simulink model "My_gfm_datacenter_BESS"  (R2018b)
settings: Solver=ode45  StartTime=0.0  StopTime=100  MaxStep=1e-4  RelTol=1e-3
PreLoadFcn:
  | modelDir = fileparts(get_param(bdroot,'FileName'));
  | 
  | load_system(fullfile(modelDir,'controls_element_lib.slx'));
  | load_system(fullfile(modelDir,'test_sequence_lib.slx'));
InitFcn:
  | close all;
  | clear all;
  | clc;
  | 
  | close all;
  | clear all;
  | clc;
  | 
  | % frequency nominals
  | F_NOM = 60;
  | W_NOM = 2 * pi * F_NOM;
  | 
  | % base values relative to inverter
  | % --------------------------------
  | VLL_INV_NOM = 34.5e3;
  | P_INV_NOM = 5e6;
  | Q_INV_NOM = 2.5e6;
  | S_INV_NOM = sqrt(P_INV_NOM^2 + Q_INV_NOM^2);
  | 
  | I_INV_BASE = S_INV_NOM/(sqrt(3)*VLL_INV_NOM);
  | Z_INV_BASE = VLL_INV_NOM^2/S_INV_NOM;
  | L_INV_BASE = Z_INV_BASE / W_NOM;
  | C_INV_BASE = 1 / (Z_INV_BASE * W_NOM);
  | 
  | % SST Parameters
  | N_DCDC_XFMR = 3;
  | N_CELLS_PER_STRING = 10;
  | C_MV_CELL = 400e-6;
  | C_LV_SST = 5e-3;
  | C_BBU = 1500; % 60 sec * 5MW
  | r_BBU = 5e-3;
  | ILV_MAX = 300;
  | ILV_MIN = -300;
  | IMV_MAX = 100;
  | IMV_MIN = -100;
  | V_LVDC_NOM = 800;
  | IDC_NOM = P_INV_NOM / V_LVDC_NOM;
  | 
  | % nominal ratings for power system model
  | % --------------------------------------
  | INVERTER_COUNT = 20;
  | 
  | VMV_NOM = VLL_INV_NOM;
  | VHV_NOM = 230e3;
  | S_PLANT = INVERTER_COUNT * S_INV_NOM;
  | 
  | N_GSU = VHV_NOM/VMV_NOM;
  | 
  | I_MV_BASE = S_PLANT/(sqrt(3)*VMV_NOM);
  | I_HV_BASE = S_PLANT/(sqrt(3)*VHV_NOM);
  | 
  | Z_MV_BASE = VMV_NOM^2/S_PLANT;
  | Z_HV_BASE = VHV_NOM^2/S_PLANT;
  | 
  | L_MV_BASE = Z_MV_BASE / W_NOM;
  | L_HV_BASE = Z_HV_BASE / W_NOM;
  | C_MV_BASE = 1 / (Z_MV_BASE * W_NOM);
  | C_HV_BASE = 1 / (Z_HV_BASE * W_NOM);
libraries: controls_element_lib x20, test_sequence_lib x13, simulink x3
settings Model: SimulationMode=accelerator  Creator=HussamAlatrash  LastModifiedBy=ahhei
settings DataIOCC: SaveOutput=off  SignalLogging=off  DSMLogging=off  SaveTime=off
settings OptimizationCC: EfficientMapNaN2IntZero=off
settings DebuggingCC: UnconnectedInputMsg=none  UnconnectedOutputMsg=none  UnconnectedLineMsg=none
settings HardwareCC: TargetBitPerPointer=64  TargetBitPerSizeT=64  TargetBitPerPtrDiffT=64  TargetLongLongMode=on  TargetIntDivRoundTo=Zero  TargetEndianess=LittleEndian  TargetWordSize=64  TargetHWDeviceType=MATLAB Host  ProdEqTarget=off
settings ModelReferenceCC: EnableRefExpFcnMdlSchedulingChecks=off
settings CodeAppCC: MaxIdLength=128
settings GRTTargetCC: TargetLangStandard=C89/C90 (ANSI)  CombineOutputUpdateFcns=off  GRTInterface=on

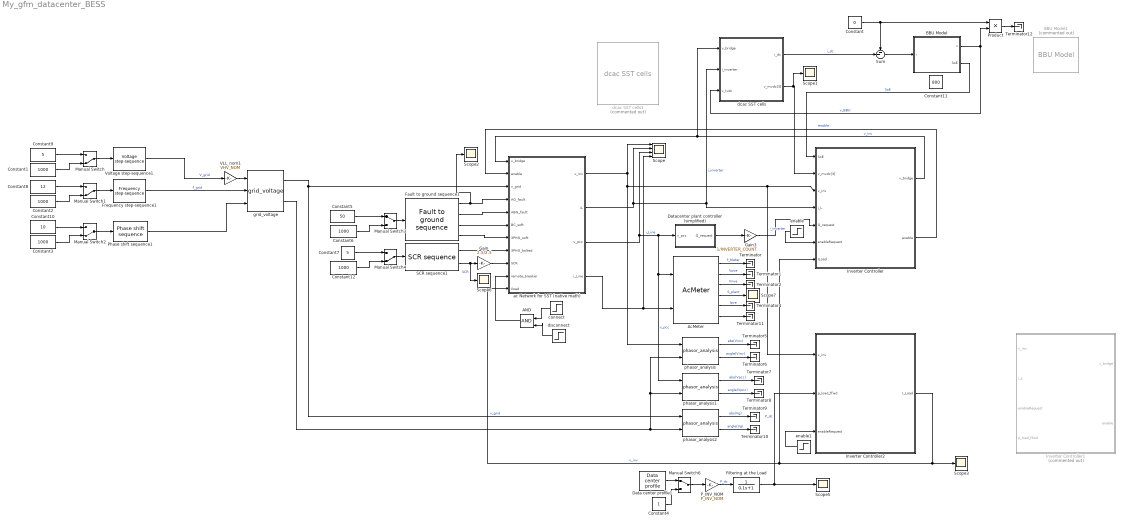
== system My_gfm_datacenter_BESS ==
  AND : Logic  IconShape=distinctive  AllPortsSameDT=off  OutDataTypeStr=boolean
  AcMeter : test_sequence_lib/AcMeter  VllRated=VHV_NOM
  BBU Model : Subsystem  AncestorBlock=test_sequence_lib/BBU Model
  BBU Model1 : test_sequence_lib/BBU Model  Commented=on  SystemSampleTime=-1
  Constant : Constant  Value=0
  Constant{1..3,6,12} (5 alike) : Constant  Value=1000
  Constant10 : Constant  Value=10
  Constant11 : Constant  Value=800
  Constant4 : Constant
  Constant5 : Constant  Value=50
  Constant7 : Constant  Value=5
  Constant8 : Constant  Value=12
  Constant9 : Constant  Value=5
  Data center profile1 : test_sequence_lib/Data center profile  SystemSampleTime=-1
  Datacenter plant controller (simplified) : Subsystem  AncestorBlock=controls_element_lib/Datacenter plant controller
  Fault to ground sequence1 : test_sequence_lib/Fault to ground sequence  SystemSampleTime=-1
  Filtering at the Load : TransferFcn  Denominator=[0.1 1]
  Frequency step-sequence1 : test_sequence_lib/Frequency step-sequence  SystemSampleTime=-1
  Gain : Gain  Gain=2.5/2.5
  Gain3 : Gain  Gain=1/INVERTER_COUNT
  Inverter Controller : Subsystem
  Inverter Controller1 : Subsystem  Commented=on
  Inverter Controller2 : Subsystem
  Manual Switch{,1..2,4} (4 alike) : ManualSwitch  CurrentSetting=0
  Manual Switch3 : ManualSwitch
  Manual Switch6 : ManualSwitch
  P_INV_NOM : Gain  Gain=P_INV_NOM
  Phase shift sequence1 : test_sequence_lib/Phase shift sequence  SystemSampleTime=-1
  Product : Product
  SCR sequence1 : test_sequence_lib/SCR sequence  SystemSampleTime=-1
  Scope : Scope  NumInputPorts=4
  Scope{1..3,5..7} (6 alike) : Scope
  Sum : Sum  Inputs=--|
  Terminator{,1..2,4..12} (12 alike) : Terminator
  VLL_nom1 : Gain  Gain=VHV_NOM
  Voltage step-sequence1 : test_sequence_lib/Voltage step-sequence  SystemSampleTime=-1
  ac Network for SST (native math) : Subsystem  AncestorBlock=test_sequence_lib/ac Network for SST (native math)
  connect : Step  Time=0  SampleTime=0
  dcac SST cells : Subsystem  AncestorBlock=test_sequence_lib/dcac SST cells
  dcac SST cells1 : test_sequence_lib/dcac SST cells  Commented=on  SystemSampleTime=-1
  disconnect : Step  Time=97  Before=1  SampleTime=0
  enable : Step  Time=2  SampleTime=0
  enable1 : Step  Time=4  SampleTime=0
  grid_voltage : test_sequence_lib/grid_voltage  SystemSampleTime=-1
  phasor_analysis : test_sequence_lib/phasor_analysis  SystemSampleTime=-1
  phasor_analysis1 : test_sequence_lib/phasor_analysis  SystemSampleTime=-1
  phasor_analysis2 : test_sequence_lib/phasor_analysis  SystemSampleTime=-1
  wires:
  Inverter Controller/2(enable) -> ac Network for SST (native math)/2(enable)  "enable"
  Constant9/1 -> Manual Switch/1
  Constant3/1 -> Manual Switch2/2
  VLL_nom1/1 -> grid_voltage/1
  Manual Switch3/1 -> Fault to ground sequence1/1
  Voltage step-sequence1/1 -> VLL_nom1/1  "V_grid"
  Constant6/1 -> Manual Switch3/2
  Fault to ground sequence1/2 -> ac Network for SST (native math)/5(ABG_fault)
  ac Network for SST (native math)/4(i_Line) -> Scope/4, AcMeter/2  "i_Line"
  ac Network for SST (native math)/1(v_inv) -> Scope/1, Inverter Controller2/1(v_inv), Inverter Controller/3(v_inv), phasor_analysis/1  "i_inverter"
  Constant8/1 -> Manual Switch1/1
  Gain/1 -> ac Network for SST (native math)/9(SCR)
  Inverter Controller/1(v_bridge) -> dcac SST cells/1(v_bridge), ac Network for SST (native math)/1(v_bridge)  "v_inv"
  SCR sequence1/2 -> Scope6/1, Gain/1  "SCR"
  phasor_analysis1/2 -> Terminator8/1  "angle(Vpcc)"
  Constant1/1 -> Manual Switch/2
  Fault to ground sequence1/1 -> Scope2/1, ac Network for SST (native math)/4(AG_fault)
  Frequency step-sequence1/1 -> grid_voltage/2  "f_grid"
  Constant5/1 -> Manual Switch3/1
  Fault to ground sequence1/4 -> ac Network for SST (native math)/7(3PHG_soft)
  Fault to ground sequence1/3 -> ac Network for SST (native math)/6(BC_soft)
  AcMeter/2 -> Terminator1/1  "Vpve"
  dcac SST cells/1(i_dc) -> Sum/2  "i_dc"
  phasor_analysis/1 -> Terminator5/1  "abs(Vinv)"
  AcMeter/4 -> Scope7/1  "S_plant"
  Manual Switch/1 -> Voltage step-sequence1/1
  Manual Switch1/1 -> Frequency step-sequence1/1
  Datacenter plant controller (simplified)/1(Q_request) -> Gain3/1
  connect/1 -> AND/1
  Phase shift sequence1/1 -> grid_voltage/3
  Constant10/1 -> Manual Switch2/1
  disconnect/1 -> AND/2
  ac Network for SST (native math)/2(iL) -> Scope/2, Inverter Controller/4(i_L), dcac SST cells/2(i_inverter)  "i_inverter"
  dcac SST cells/2(v_mvdc[3]) -> Scope1/1, Inverter Controller/2(v_mvdc[3])
  AND/1 -> ac Network for SST (native math)/10(remote_breaker)
  enable/1 -> Inverter Controller/6(enableRequest)
  Constant7/1 -> Manual Switch4/1
  grid_voltage/2 -> phasor_analysis1/2, phasor_analysis/2, phasor_analysis2/2
  grid_voltage/1 -> phasor_analysis2/1, ac Network for SST (native math)/3(v_grid)  "v_grid"
  SCR sequence1/1 -> ac Network for SST (native math)/8(3PHG_bolted)
  phasor_analysis1/1 -> Terminator7/1  "abs(Vpcc)"
  ac Network for SST (native math)/3(v_pcc) -> Scope/3, Datacenter plant controller (simplified)/1(v_pcc), phasor_analysis1/1, AcMeter/1  "v_pcc"
  Constant12/1 -> Manual Switch4/2
  BBU Model/1(v) -> dcac SST cells/3(v_lvdc), Product/2  "v_BBU"
  Constant/1 -> Sum/1, Product/1
  phasor_analysis2/2 -> Terminator10/1  "angle(Vg)"
  BBU Model/2(SoE) -> Inverter Controller/1(SoE)  "SoE"
  Gain3/1 -> Inverter Controller/5(Q_request)
  phasor_analysis/2 -> Terminator6/1  "angle(Vinv)"
  AcMeter/3 -> Terminator2/1  "Vnve"
  AcMeter/5 -> Terminator4/1  "Ipve"
  Constant2/1 -> Manual Switch1/2
  phasor_analysis2/1 -> Terminator9/1  "abs(Vg)"
  Manual Switch4/1 -> SCR sequence1/1
  Sum/1 -> BBU Model/1(i)
  AcMeter/6 -> Terminator11/1
  AcMeter/1 -> Terminator/1  "f_Meter"
  Manual Switch2/1 -> Phase shift sequence1/1
  enable1/1 -> Inverter Controller2/3(enableRequest)
  Inverter Controller2/1(I_Load) -> Inverter Controller/7(ILoad), ac Network for SST (native math)/11(Iload), Scope3/1  "v_inv"
  Manual Switch6/1 -> P_INV_NOM/1
  Data center profile1/1 -> Manual Switch6/1
  Constant4/1 -> Manual Switch6/2
  P_INV_NOM/1 -> Filtering at the Load/1  "P_dc"
  Product/1 -> Terminator12/1
  Filtering at the Load/1 -> Inverter Controller2/2(p_load_ffwd), Scope5/1  "P_dc"

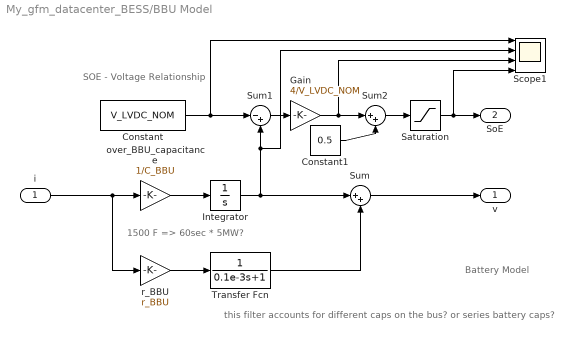
== system My_gfm_datacenter_BESS/BBU Model ==
  note: Battery Model
  note: this filter accounts for different caps on the bus? or series battery caps?
  note: 1500 F => 60sec * 5MW?
  note: SOE - Voltage Relationship
  i : Inport
  Constant : Constant  Value=V_LVDC_NOM
  Constant1 : Constant  Value=0.5
  Gain : Gain  Gain=4/V_LVDC_NOM
  Integrator : Integrator  InitialCondition=V_LVDC_NOM
  Saturation : Saturate  UpperLimit=1.1  LowerLimit=-0.1
  Scope1 : Scope  NumInputPorts=4
  Sum : Sum  Inputs=|++
  Sum1 : Sum  Inputs=|-+
  Sum2 : Sum  Inputs=|++
  Transfer Fcn : TransferFcn  Denominator=[0.1e-3 1]
  over_BBU_capacitance : Gain  Gain=1/C_BBU
  r_BBU : Gain  Gain=r_BBU
  v : Outport  VectorParamsAs1DForOutWhenUnconnected=on
  SoE : Outport  Port=2  VectorParamsAs1DForOutWhenUnconnected=on
  wires:
  Saturation/1 -> Scope1/4, SoE/1
  Constant1/1 -> Sum2/2
  Sum2/1 -> Saturation/1
  Constant/1 -> Scope1/1, Sum1/1
  Sum1/1 -> Gain/1
  Gain/1 -> Scope1/3, Sum2/1
  Transfer Fcn/1 -> Sum/2
  Sum/1 -> v/1
  r_BBU/1 -> Transfer Fcn/1
  i/1 -> over_BBU_capacitance/1, r_BBU/1
  Integrator/1 -> Scope1/2, Sum1/2, Sum/1
  over_BBU_capacitance/1 -> Integrator/1

== system My_gfm_datacenter_BESS/Datacenter plant controller (simplified) ==
  v_pcc : Inport
  Gain4 : Gain  Gain=1/VHV_NOM
  Meter : Subsystem
  SRated2 : Gain  Gain=S_PLANT
  VoltVAr : Subsystem
  Q_request : Outport  VectorParamsAs1DForOutWhenUnconnected=on
  wires:
  v_pcc/1 -> Gain4/1
  SRated2/1 -> Q_request/1  "Q_request"
  Meter/1(V_estimate) -> VoltVAr/1(V)  "V_pu_plant"
  Gain4/1 -> Meter/1(v)
  VoltVAr/1(Q) -> SRated2/1

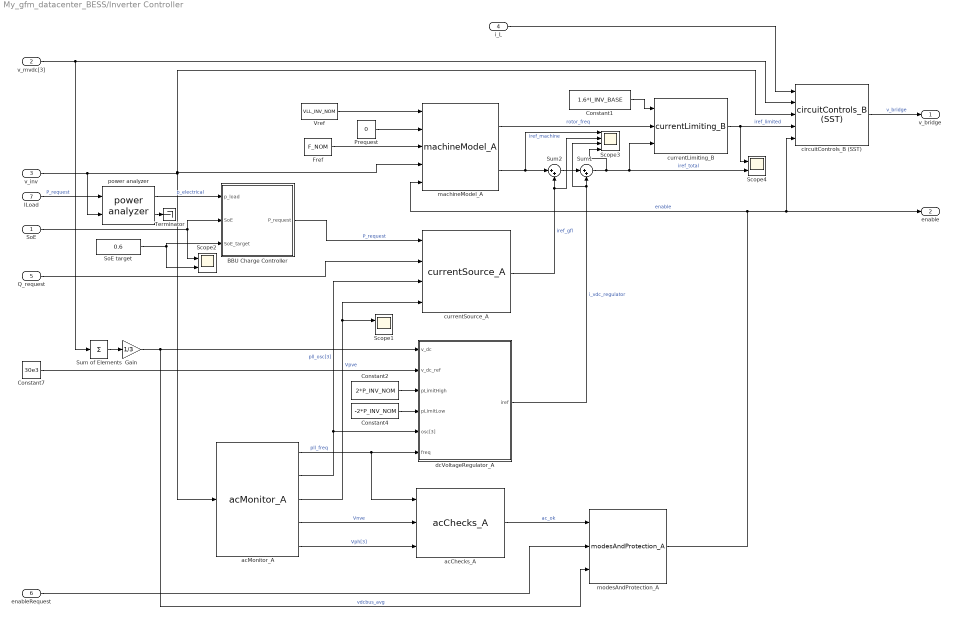
== system My_gfm_datacenter_BESS/Inverter Controller ==
  SoE : Inport
  v_mvdc[3] : Inport  Port=2
  v_inv : Inport  Port=3
  i_L : Inport  Port=4
  Q_request : Inport  Port=5
  enableRequest : Inport  Port=6
  ILoad : Inport  Port=7
  BBU Charge Controller : Subsystem  AncestorBlock=controls_element_lib/BBU Charge Controller
  Constant1 : Constant  Value=1.6*I_INV_BASE
  Constant2 : Constant  Value=2*P_INV_NOM
  Constant4 : Constant  Value=-2*P_INV_NOM
  Constant7 : Constant  Value=30e3
  Fref : Constant  Value=F_NOM
  Gain : Gain  Gain=1/3
  Prequest : Constant  Value=0
  Scope1 : Scope  NumInputPorts=2
  Scope2 : Scope  NumInputPorts=2
  Scope3 : Scope  NumInputPorts=4
  Scope4 : Scope  NumInputPorts=2
  SoE target : Constant  Value=0.6
  Sum of Elements : Sum  Inputs=+
  Sum1 : Sum  Inputs=|++
  Sum2 : Sum  Inputs=|++
  Terminator : Terminator
  Vref : Constant  Value=VLL_INV_NOM
  acChecks_A : controls_element_lib/acChecks_A  VllRated=VLL_INV_NOM  nominalFrequency=F_NOM  tRequalify=2  T_CNTL=1e-3
  acMonitor_A : controls_element_lib/acMonitor_A  VllRated=VLL_INV_NOM  nominalFrequency=F_NOM
  circuitControls_B (SST) : controls_element_lib/circuitControls_B (SST)  SystemSampleTime=-1
  currentLimiting_B : controls_element_lib/currentLimiting_B  IRated=I_INV_BASE  peakSoftLimit=2.6  peakHardLimit=3.6
  currentSource_A : controls_element_lib/currentSource_A  VllRated=VLL_INV_NOM  SRated=S_INV_NOM  nominalFrequency=F_NOM  Plimit=P_INV_NOM/S_INV_NOM  Qlimit=Q_INV_NOM/S_INV_NOM
  dcVoltageRegulator_A : Subsystem  AncestorBlock=controls_element_lib/dcVoltageRegulator_A  mask{kp=0.5e3, kSlowPath=5e3, wSlowPath=5, pLimitExternalMinimum=0.05*P_INV_NOM, vdc_deadband=1500, VllRated=VLL_INV_NOM}
      mask prompts: kp "Proportional gain (W/V)"; kSlowPath "Slow path gain (W/V)"; wSlowPath "Slow path bandwidth (rad)"; pLimitExternalMinimum "Minimum value for external power limit (W)"; vdc_deadband "Deadband around reference voltage (V)"; VllRated "Rated Voltage (Volts, line-to-line)"
  machineModel_A : controls_element_lib/machineModel_A  SRated=S_INV_NOM  VllRated=VLL_INV_NOM  nominalFrequency=F_NOM  inertialConstant=2.5  kDroop=0  kDamper=1  Xs=0.1  rs=0.08  Qlimit=0.5  wExciter=10
  modesAndProtection_A : controls_element_lib/modesAndProtection_A  dcOvervotlageThreshold=40e3  dcUndervotlageThreshold=23e3  dcTripClearTimeout=0.2
  power analyzer : controls_element_lib/machineModel_A/power analyzer  SystemSampleTime=-1
  v_bridge : Outport  VectorParamsAs1DForOutWhenUnconnected=on
  enable : Outport  Port=2  VectorParamsAs1DForOutWhenUnconnected=on
  wires:
  Vref/1 -> machineModel_A/1
  Prequest/1 -> machineModel_A/2
  Fref/1 -> machineModel_A/3
  machineModel_A/2 -> Scope3/1, Sum2/1  "iref_machine"
  currentLimiting_B/1 -> Scope4/1, circuitControls_B (SST)/4  "iref_limited"
  v_inv/1 -> power analyzer/2, circuitControls_B (SST)/3, machineModel_A/4, acMonitor_A/1
  currentSource_A/1 -> Scope3/2, Sum2/2  "iref_gfl"
  Sum1/1 -> Scope3/4, Scope4/2, currentLimiting_B/3  "iref_total"
  acMonitor_A/2 -> currentSource_A/3, dcVoltageRegulator_A/5(osc[3])  "pll_osc[3]"
  Q_request/1 -> currentSource_A/2
  acMonitor_A/4 -> acChecks_A/2  "Vnve"
  enableRequest/1 -> modesAndProtection_A/2
  modesAndProtection_A/1 -> machineModel_A/5, enable/1, circuitControls_B (SST)/5  "enable"
  acMonitor_A/3 -> Scope1/1, currentSource_A/4  "Vpve"
  Constant1/1 -> currentLimiting_B/1
  acMonitor_A/5 -> acChecks_A/3  "Vph[3]"
  acChecks_A/1 -> modesAndProtection_A/1  "ac_ok"
  acMonitor_A/1 -> dcVoltageRegulator_A/6(freq), acChecks_A/1  "pll_freq"
  dcVoltageRegulator_A/1(iref) -> Scope3/3, Sum1/2  "i_vdc_regulator"
  Sum2/1 -> Sum1/1
  Constant7/1 -> dcVoltageRegulator_A/2(v_dc_ref)
  Sum of Elements/1 -> Gain/1
  Gain/1 -> modesAndProtection_A/3, dcVoltageRegulator_A/1(v_dc)  "vdcbus_avg"
  Constant2/1 -> dcVoltageRegulator_A/3(pLimitHigh)
  Constant4/1 -> dcVoltageRegulator_A/4(pLimitLow)
  SoE/1 -> Scope2/1, BBU Charge Controller/2(SoE)
  circuitControls_B (SST)/1 -> v_bridge/1  "v_bridge"
  v_mvdc[3]/1 -> Sum of Elements/1, circuitControls_B (SST)/2
  i_L/1 -> circuitControls_B (SST)/1
  SoE target/1 -> BBU Charge Controller/3(SoE_target), Scope2/2
  machineModel_A/1 -> currentLimiting_B/2  "rotor_freq"
  BBU Charge Controller/1(P_request) -> currentSource_A/1  "P_request"
  ILoad/1 -> power analyzer/1  "P_request"
  power analyzer/1 -> BBU Charge Controller/1(p_load)  "p_electrical"
  power analyzer/2 -> Terminator/1

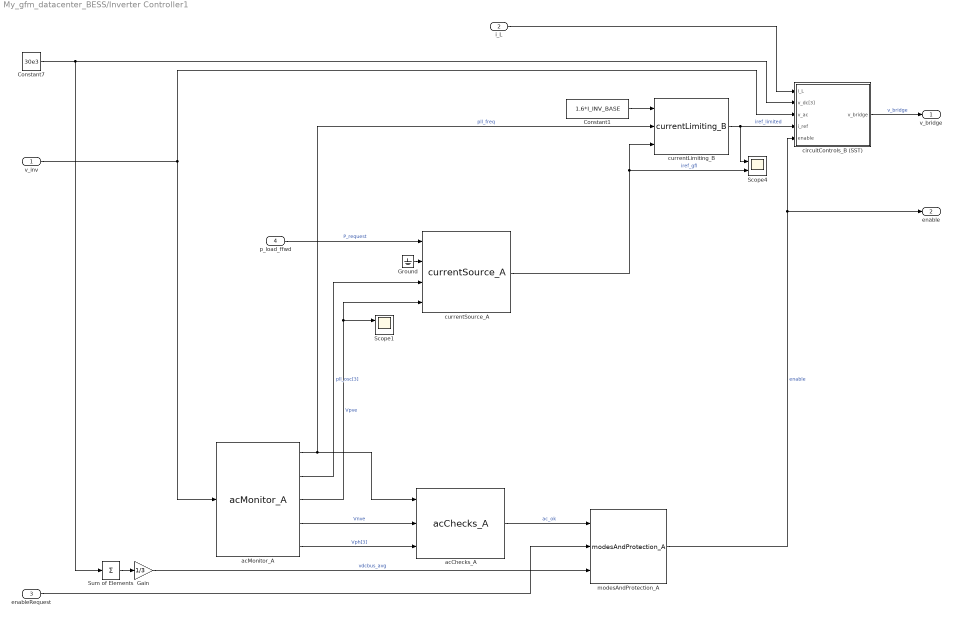
== system My_gfm_datacenter_BESS/Inverter Controller1 ==
  v_inv : Inport
  i_L : Inport  Port=2
  enableRequest : Inport  Port=3
  p_load_ffwd : Inport  Port=4
  Constant1 : Constant  Value=1.6*I_INV_BASE
  Constant7 : Constant  Value=30e3
  Gain : Gain  Gain=1/3
  Ground : Ground
  Scope1 : Scope  NumInputPorts=2
  Scope4 : Scope  NumInputPorts=2
  Sum of Elements : Sum  Inputs=+
  acChecks_A : controls_element_lib/acChecks_A  VllRated=VLL_INV_NOM  nominalFrequency=F_NOM  tRequalify=2  T_CNTL=1e-3
  acMonitor_A : controls_element_lib/acMonitor_A  VllRated=VLL_INV_NOM  nominalFrequency=F_NOM
  circuitControls_B (SST) : Subsystem  AncestorBlock=controls_element_lib/circuitControls_B (SST)
  currentLimiting_B : controls_element_lib/currentLimiting_B  IRated=I_INV_BASE  peakSoftLimit=2.6  peakHardLimit=3.6
  currentSource_A : controls_element_lib/currentSource_A  VllRated=VLL_INV_NOM  SRated=S_INV_NOM  nominalFrequency=F_NOM  Plimit=P_INV_NOM/S_INV_NOM  Qlimit=Q_INV_NOM/S_INV_NOM
  modesAndProtection_A : controls_element_lib/modesAndProtection_A  dcOvervotlageThreshold=40e3  dcUndervotlageThreshold=23e3  dcTripClearTimeout=0.2
  v_bridge : Outport  VectorParamsAs1DForOutWhenUnconnected=on
  enable : Outport  Port=2  VectorParamsAs1DForOutWhenUnconnected=on
  wires:
  currentLimiting_B/1 -> Scope4/1, circuitControls_B (SST)/4(i_ref)  "iref_limited"
  v_inv/1 -> circuitControls_B (SST)/3(v_ac), acMonitor_A/1
  currentSource_A/1 -> Scope4/2, currentLimiting_B/3  "iref_gfl"
  acMonitor_A/2 -> currentSource_A/3  "pll_osc[3]"
  acMonitor_A/4 -> acChecks_A/2  "Vnve"
  enableRequest/1 -> modesAndProtection_A/2
  modesAndProtection_A/1 -> enable/1, circuitControls_B (SST)/5(enable)  "enable"
  p_load_ffwd/1 -> currentSource_A/1  "P_request"
  acMonitor_A/3 -> Scope1/1, currentSource_A/4  "Vpve"
  Constant1/1 -> currentLimiting_B/1
  acMonitor_A/5 -> acChecks_A/3  "Vph[3]"
  acChecks_A/1 -> modesAndProtection_A/1  "ac_ok"
  acMonitor_A/1 -> currentLimiting_B/2, acChecks_A/1  "pll_freq"
  Sum of Elements/1 -> Gain/1
  Gain/1 -> modesAndProtection_A/3  "vdcbus_avg"
  circuitControls_B (SST)/1(v_bridge) -> v_bridge/1  "v_bridge"
  Constant7/1 -> Sum of Elements/1, circuitControls_B (SST)/2(v_dc[3])
  i_L/1 -> circuitControls_B (SST)/1(i_L)
  Ground/1 -> currentSource_A/2

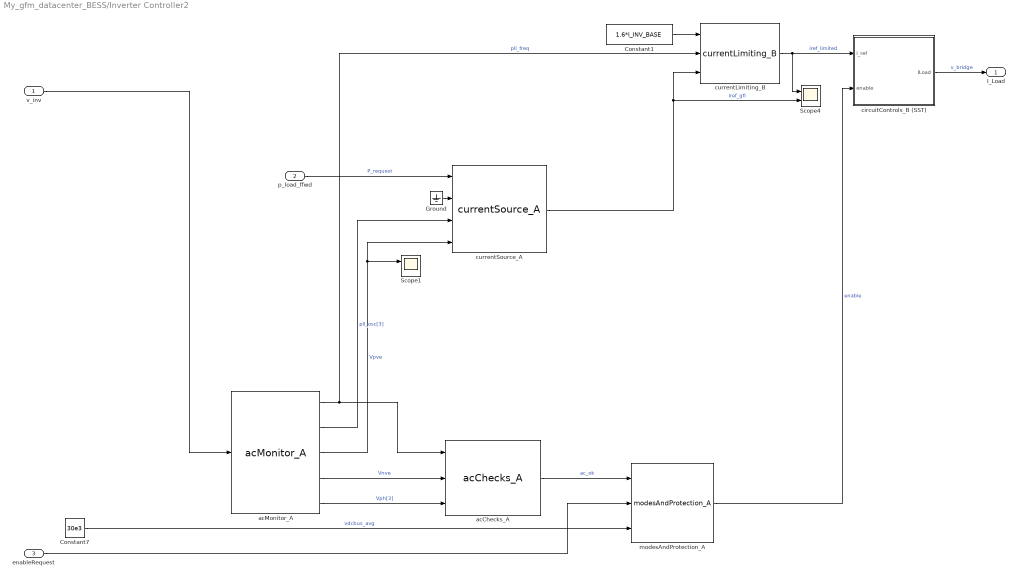
== system My_gfm_datacenter_BESS/Inverter Controller2 ==
  v_inv : Inport
  p_load_ffwd : Inport  Port=2
  enableRequest : Inport  Port=3
  Constant1 : Constant  Value=1.6*I_INV_BASE
  Constant7 : Constant  Value=30e3
  Ground : Ground
  Scope1 : Scope  NumInputPorts=2
  Scope4 : Scope  NumInputPorts=2
  acChecks_A : controls_element_lib/acChecks_A  VllRated=VLL_INV_NOM  nominalFrequency=F_NOM  tRequalify=2  T_CNTL=1e-3
  acMonitor_A : controls_element_lib/acMonitor_A  VllRated=VLL_INV_NOM  nominalFrequency=F_NOM
  circuitControls_B (SST) : Subsystem  AncestorBlock=controls_element_lib/circuitControls_B (SST)
  currentLimiting_B : controls_element_lib/currentLimiting_B  IRated=I_INV_BASE  peakSoftLimit=2.6  peakHardLimit=3.6
  currentSource_A : controls_element_lib/currentSource_A  VllRated=VLL_INV_NOM  SRated=S_INV_NOM  nominalFrequency=F_NOM  Plimit=P_INV_NOM/S_INV_NOM  Qlimit=Q_INV_NOM/S_INV_NOM
  modesAndProtection_A : controls_element_lib/modesAndProtection_A  dcOvervotlageThreshold=40e3  dcUndervotlageThreshold=23e3  dcTripClearTimeout=0.2
  I_Load : Outport  VectorParamsAs1DForOutWhenUnconnected=on
  wires:
  currentLimiting_B/1 -> Scope4/1, circuitControls_B (SST)/1(i_ref)  "iref_limited"
  v_inv/1 -> acMonitor_A/1
  currentSource_A/1 -> Scope4/2, currentLimiting_B/3  "iref_gfl"
  acMonitor_A/2 -> currentSource_A/3  "pll_osc[3]"
  acMonitor_A/4 -> acChecks_A/2  "Vnve"
  enableRequest/1 -> modesAndProtection_A/2
  modesAndProtection_A/1 -> circuitControls_B (SST)/2(enable)  "enable"
  p_load_ffwd/1 -> currentSource_A/1  "P_request"
  acMonitor_A/3 -> Scope1/1, currentSource_A/4  "Vpve"
  Constant1/1 -> currentLimiting_B/1
  acMonitor_A/5 -> acChecks_A/3  "Vph[3]"
  acChecks_A/1 -> modesAndProtection_A/1  "ac_ok"
  acMonitor_A/1 -> currentLimiting_B/2, acChecks_A/1  "pll_freq"
  Constant7/1 -> modesAndProtection_A/3  "vdcbus_avg"
  circuitControls_B (SST)/1(ILoad) -> I_Load/1  "v_bridge"
  Ground/1 -> currentSource_A/2

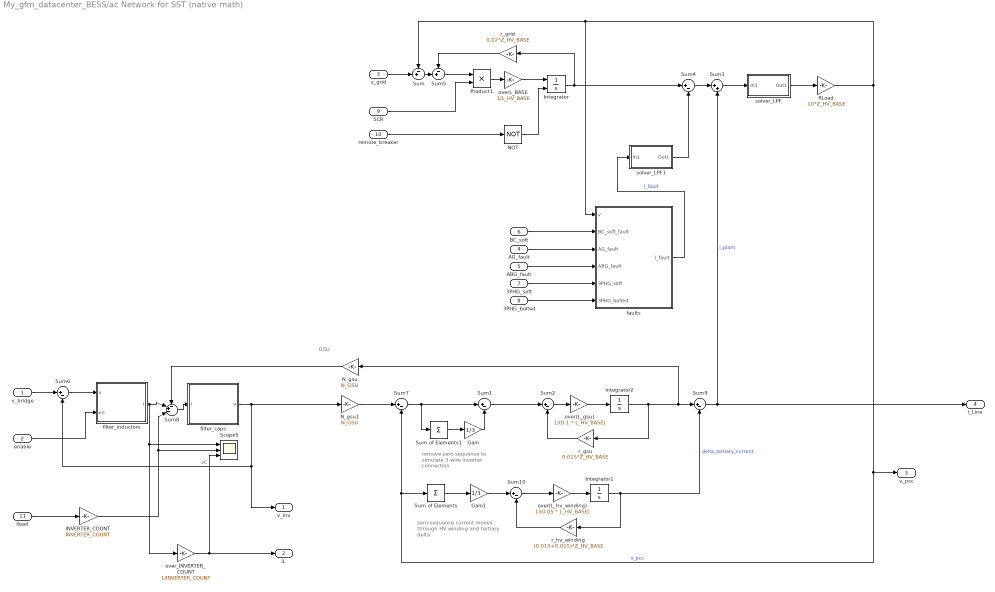
== system My_gfm_datacenter_BESS/ac Network for SST (native math) ==
  note: zero-sequence current moves through HV winding and tertiary delta
  note: remove zero-sequence to simulate 3-wire inverter connection
  note: GSU
  v_bridge : Inport
  enable : Inport  Port=2
  v_grid : Inport  Port=3
  AG_fault : Inport  Port=4
  ABG_fault : Inport  Port=5
  BC_soft : Inport  Port=6
  3PHG_soft : Inport  Port=7
  3PHG_bolted : Inport  Port=8
  SCR : Inport  Port=9
  remote_breaker : Inport  Port=10
  Iload : Inport  Port=11
  Gain : Gain  Gain=1/3
  Gain1 : Gain  Gain=1/3
  INVERTER_COUNT : Gain  Gain=INVERTER_COUNT
  Integrator : Integrator  ExternalReset=level
  Integrator1 : Integrator
  Integrator2 : Integrator
  NOT : Logic  Operator=NOT  IconShape=distinctive  AllPortsSameDT=off  OutDataTypeStr=boolean
  N_gsu : Gain  Gain=N_GSU
  N_gsu1 : Gain  Gain=N_GSU
  Product1 : Product
  RLoad : Gain  Gain=10*Z_HV_BASE
  Scope5 : Scope  NumInputPorts=3
  Sum : Sum  Inputs=-+|
  Sum of Elements : Sum  Inputs=+
  Sum of Elements1 : Sum  Inputs=+
  Sum{1..2,4,6..7,9..10} (7 alike) : Sum  Inputs=|+-
  Sum3 : Sum  Inputs=|++
  Sum5 : Sum  Inputs=-+|
  Sum8 : Sum  Inputs=-+-|
  faults : Subsystem
  filter_caps : Subsystem
  filter_inductors : Subsystem
  over(L_gsu) : Gain  Gain=1/(0.1 * L_HV_BASE)
  over(L_hv_winding) : Gain  Gain=1/(0.05 * L_HV_BASE)
  overL_BASE : Gain  Gain=1/L_HV_BASE
  over_INVERTER_COUNT : Gain  Gain=1/INVERTER_COUNT
  r_grid : Gain  Gain=0.02*Z_HV_BASE
  r_gsu : Gain  Gain=0.015*Z_HV_BASE
  r_hv_winding : Gain  Gain=(0.015+0.015)*Z_HV_BASE
  solver_LPF : Subsystem
  solver_LPF1 : Subsystem
  v_inv : Outport  VectorParamsAs1DForOutWhenUnconnected=on
  iL : Outport  Port=2  VectorParamsAs1DForOutWhenUnconnected=on
  v_pcc : Outport  Port=3  VectorParamsAs1DForOutWhenUnconnected=on
  i_Line : Outport  Port=4  VectorParamsAs1DForOutWhenUnconnected=on
  wires:
  AG_fault/1 -> faults/3(AG_fault)
  ABG_fault/1 -> faults/4(ABG_fault)
  BC_soft/1 -> faults/2(BC_soft_fault)
  Gain1/1 -> Sum10/1
  Sum of Elements/1 -> Gain1/1
  Sum10/1 -> over(L_hv_winding)/1
  r_hv_winding/1 -> Sum10/2
  Integrator1/1 -> r_hv_winding/1, Sum9/2  "delta_tertiary_current"
  over(L_hv_winding)/1 -> Integrator1/1
  Sum9/1 -> i_Line/1, Sum3/2  "i_plant"
  N_gsu1/1 -> Sum7/1
  over_INVERTER_COUNT/1 -> Scope5/3, iL/1
  filter_caps/1(v) -> N_gsu1/1, Sum6/2, v_inv/1  "vC"
  Sum8/1 -> filter_caps/1(i)
  filter_inductors/1(i) -> Scope5/1, over_INVERTER_COUNT/1, Sum8/2
  enable/1 -> filter_inductors/2(en)
  Sum6/1 -> filter_inductors/1(v)
  r_gsu/1 -> Sum2/2
  Sum1/1 -> Sum2/1
  Gain/1 -> Sum1/2
  Sum of Elements1/1 -> Gain/1
  Sum2/1 -> over(L_gsu)/1
  Sum7/1 -> Sum1/1, Sum of Elements1/1
  over(L_gsu)/1 -> Integrator2/1
  solver_LPF/1(Out1) -> RLoad/1
  remote_breaker/1 -> NOT/1
  overL_BASE/1 -> Integrator/1
  Integrator/1 -> Sum4/1, r_grid/1
  solver_LPF1/1(Out1) -> Sum4/2
  RLoad/1 -> faults/1(v), Sum/1, v_pcc/1, Sum of Elements/1, Sum7/2  "v_pcc"
  faults/1(i_fault) -> solver_LPF1/1(In1)  "i_fault"
  3PHG_bolted/1 -> faults/6(3PHG_bolted)
  v_bridge/1 -> Sum6/1
  Product1/1 -> overL_BASE/1
  SCR/1 -> Product1/2
  r_grid/1 -> Sum5/1
  Sum3/1 -> solver_LPF/1(In1)
  NOT/1 -> Integrator/2
  Sum4/1 -> Sum3/1
  v_grid/1 -> Sum/2
  Sum5/1 -> Product1/1
  Sum/1 -> Sum5/2
  Integrator2/1 -> Sum9/1, N_gsu/1, r_gsu/1
  3PHG_soft/1 -> faults/5(3PHG_soft)
  Iload/1 -> INVERTER_COUNT/1
  INVERTER_COUNT/1 -> Scope5/2, Sum8/3
  N_gsu/1 -> Sum8/1

== system My_gfm_datacenter_BESS/dcac SST cells ==
  note: Should be divided by Ncells_per phase?
  note: The three aggregate dc-bus voltages for the three phases do not naturally balance and need this algorithm to do so
  note: Multiplied by Ncells_per phase
  note: Which is the command?
  note: Is it real and when is it needed?
  note: Are these real component values
  v_bridge : Inport
  i_inverter : Inport  Port=2
  v_lvdc : Inport  Port=3
  Gain1 : Gain  Gain=1/3
  N_cells : Gain  Gain=N_CELLS_PER_STRING
  N_cells1 : Gain  Gain=N_CELLS_PER_STRING
  SST Cell Model : Subsystem
  Sum of Elements : Sum  Inputs=+
  Sum of Elements1 : Sum  Inputs=+
  Sum4 : Sum  Inputs=-+|
  dcdcController : Subsystem
  kRebalance : Gain  Gain=5
  over_N_cells : Gain  Gain=1/N_CELLS_PER_STRING
  i_dc : Outport  VectorParamsAs1DForOutWhenUnconnected=on
  v_mvdc[3] : Outport  Port=2  VectorParamsAs1DForOutWhenUnconnected=on
  wires:
  i_inverter/1 -> SST Cell Model/4(i_ac)
  Sum of Elements/1 -> i_dc/1  "I_dc_sst"
  v_bridge/1 -> over_N_cells/1
  v_lvdc/1 -> dcdcController/1(v_LV), SST Cell Model/1(v_LV)
  over_N_cells/1 -> SST Cell Model/3(v_ac)
  SST Cell Model/1(v_MV_cell) -> dcdcController/2(v_MV_cell), N_cells/1  "v_mvdc_cell"
  Gain1/1 -> Sum4/2
  dcdcController/1(i_MV_ref) -> SST Cell Model/2(i_MV)
  Sum of Elements1/1 -> Gain1/1
  SST Cell Model/2(i_LV) -> N_cells1/1
  N_cells/1 -> Sum of Elements1/1, Sum4/1, v_mvdc[3]/1  "v_mvdc_bus"
  N_cells1/1 -> Sum of Elements/1
  kRebalance/1 -> dcdcController/3(P_dcdc_ffwd)  "p_string_rebalance"

== system My_gfm_datacenter_BESS/Datacenter plant controller (simplified)/Meter ==
  v : Inport
  Complex to Real-Imag : ComplexToRealImag
  Conj : Math  Operator=conj  SaturateOnIntegerOverflow=on
  Gain : Gain  Gain=sqrt(2)
  Gain1 : Gain  Gain=1/3
  Gain2 : Gain  Gain=sqrt(3)
  PLL-analog : Subsystem
  Product3 : Product
  Real-Imag to Complex : RealImagToComplex
  Sum of Elements1 : Sum  Inputs=+
  Transfer Fcn : TransferFcn  Denominator=[0.05 1]
  Transfer Fcn1 : TransferFcn  Denominator=[0.05 1]
  V_estimate : Outport  VectorParamsAs1DForOutWhenUnconnected=on
  wires:
  Gain2/1 -> V_estimate/1
  Gain1/1 -> Complex to Real-Imag/1
  Gain/1 -> Product3/2
  Real-Imag to Complex/1 -> Gain2/1
  Conj/1 -> Gain/1
  PLL-analog/2(osc) -> Conj/1
  Complex to Real-Imag/1 -> Transfer Fcn/1
  v/1 -> Product3/1, PLL-analog/1(ref)
  Complex to Real-Imag/2 -> Transfer Fcn1/1
  Product3/1 -> Sum of Elements1/1
  Transfer Fcn/1 -> Real-Imag to Complex/1
  Sum of Elements1/1 -> Gain1/1
  Transfer Fcn1/1 -> Real-Imag to Complex/2

== system My_gfm_datacenter_BESS/Datacenter plant controller (simplified)/VoltVAr ==
  V : Inport
  Abs : Abs
  Complex to Real-Imag : ComplexToRealImag
  Constant1 : Constant
  Gain : Gain  Gain=6
  Saturation : Saturate
  Sum1 : Sum  Inputs=|+-
  Transfer Fcn : TransferFcn  Denominator=[0.05 1]
  Q : Outport  VectorParamsAs1DForOutWhenUnconnected=on
  wires:
  Complex to Real-Imag/1 -> ?
  Transfer Fcn/1 -> Q/1
  Saturation/1 -> Transfer Fcn/1
  V/1 -> Abs/1, Complex to Real-Imag/1
  Abs/1 -> Sum1/2
  Constant1/1 -> Sum1/1
  Sum1/1 -> Gain/1
  Gain/1 -> Saturation/1

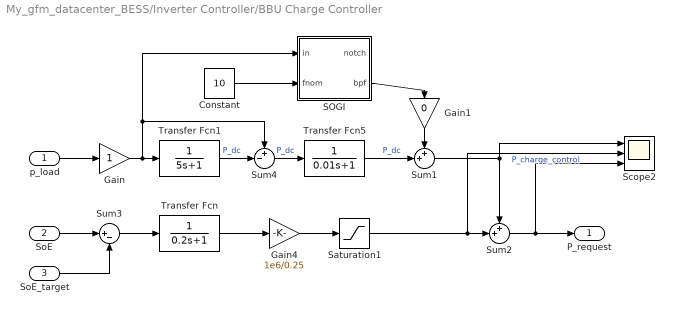
== system My_gfm_datacenter_BESS/Inverter Controller/BBU Charge Controller ==
  p_load : Inport
  SoE : Inport  Port=2
  SoE_target : Inport  Port=3
  Constant : Constant  Value=10
  Gain : Gain
  Gain1 : Gain  Gain=0
  Gain4 : Gain  Gain=1e6/0.25
  SOGI : Subsystem
  Saturation1 : Saturate  UpperLimit=P_INV_NOM  LowerLimit=-P_INV_NOM
  Scope2 : Scope  NumInputPorts=3
  Sum1 : Sum  Inputs=++|
  Sum2 : Sum  Inputs=++|
  Sum3 : Sum  Inputs=|+-
  Sum4 : Sum  Inputs=+-|
  Transfer Fcn : TransferFcn  Denominator=[0.2 1]
  Transfer Fcn1 : TransferFcn  Denominator=[5 1]
  Transfer Fcn5 : TransferFcn  Denominator=[0.01 1]
  P_request : Outport  VectorParamsAs1DForOutWhenUnconnected=on
  wires:
  Transfer Fcn/1 -> Gain4/1
  p_load/1 -> Gain/1
  Sum2/1 -> Scope2/3, P_request/1
  Gain4/1 -> Saturation1/1
  Sum4/1 -> Transfer Fcn5/1  "P_dc"
  SoE_target/1 -> Sum3/2
  Sum3/1 -> Transfer Fcn/1
  Saturation1/1 -> Sum2/2, Scope2/2  "P_charge_control"
  SoE/1 -> Sum3/1
  Gain/1 -> Sum4/1, SOGI/1(in), Transfer Fcn1/1
  Constant/1 -> SOGI/2(fnom)
  SOGI/2(bpf) -> Gain1/1
  Transfer Fcn1/1 -> Sum4/2  "P_dc"
  Sum1/1 -> Sum2/1, Scope2/1
  Transfer Fcn5/1 -> Sum1/2  "P_dc"
  Gain1/1 -> Sum1/1

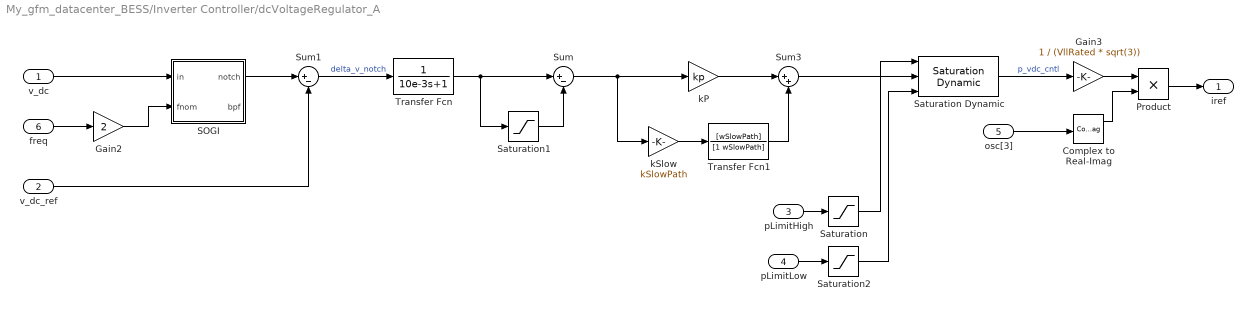
== system My_gfm_datacenter_BESS/Inverter Controller/dcVoltageRegulator_A ==
  v_dc : Inport
  v_dc_ref : Inport  Port=2
  pLimitHigh : Inport  Port=3
  pLimitLow : Inport  Port=4
  osc[3] : Inport  Port=5
  freq : Inport  Port=6
  Complex to Real-Imag : ComplexToRealImag
  Gain2 : Gain  Gain=2
  Gain3 : Gain  Gain=1 / (VllRated * sqrt(3))
  Product : Product
  SOGI : Subsystem
  Saturation : Saturate  UpperLimit=inf  LowerLimit=pLimitExternalMinimum
  Saturation Dynamic : simulink/Discontinuities/Saturation Dynamic  OutMin=[]  OutMax=[]  OutDataTypeStr=Inherit: Same as second input  OutDataType=fixdt(1, 16)  OutScaling=2^-10  DoSatur=off
  Saturation1 : Saturate  UpperLimit=vdc_deadband  LowerLimit=-vdc_deadband
  Saturation2 : Saturate  UpperLimit=-pLimitExternalMinimum  LowerLimit=-inf
  Sum : Sum  Inputs=|+-
  Sum1 : Sum  Inputs=|+-
  Sum3 : Sum  Inputs=|++
  Transfer Fcn : TransferFcn  Denominator=[10e-3 1]
  Transfer Fcn1 : TransferFcn  Numerator=[wSlowPath]  Denominator=[1 wSlowPath]
  kP : Gain  Gain=kp
  kSlow : Gain  Gain=kSlowPath
  iref : Outport  VectorParamsAs1DForOutWhenUnconnected=on
  wires:
  pLimitHigh/1 -> Saturation/1
  pLimitLow/1 -> Saturation2/1
  Transfer Fcn1/1 -> Sum3/2
  Saturation1/1 -> Sum/2
  osc[3]/1 -> Complex to Real-Imag/1
  Product/1 -> iref/1
  Gain3/1 -> Product/1
  Complex to Real-Imag/1 -> Product/2
  Gain2/1 -> SOGI/2(fnom)
  freq/1 -> Gain2/1
  v_dc/1 -> SOGI/1(in)
  SOGI/1(notch) -> Sum1/1
  Transfer Fcn/1 -> Saturation1/1, Sum/1
  Saturation Dynamic/1 -> Gain3/1  "p_vdc_cntl"
  v_dc_ref/1 -> Sum1/2
  Sum1/1 -> Transfer Fcn/1  "delta_v_notch"
  Sum/1 -> kP/1, kSlow/1
  kP/1 -> Sum3/1
  Sum3/1 -> Saturation Dynamic/2
  kSlow/1 -> Transfer Fcn1/1
  Saturation/1 -> Saturation Dynamic/1
  Saturation2/1 -> Saturation Dynamic/3

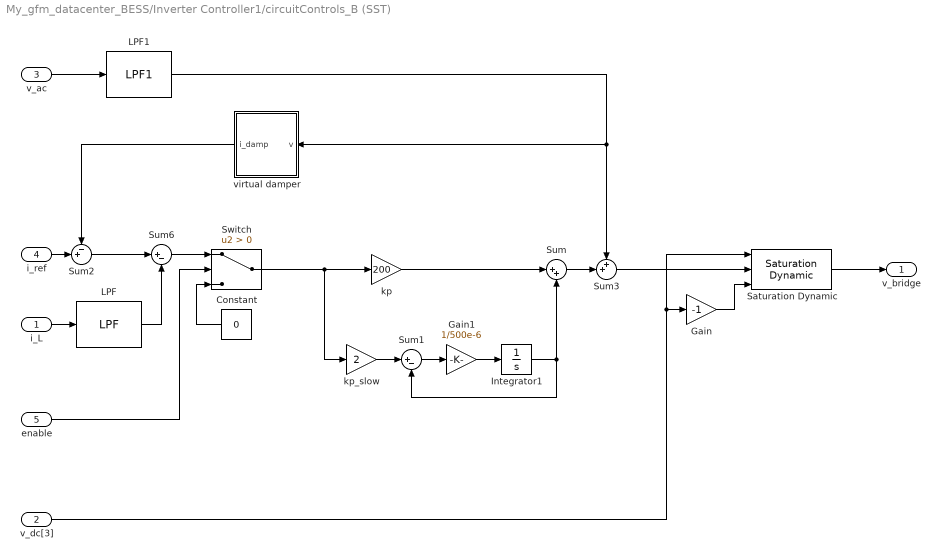
== system My_gfm_datacenter_BESS/Inverter Controller1/circuitControls_B (SST) ==
  i_L : Inport
  v_dc[3] : Inport  Port=2
  v_ac : Inport  Port=3
  i_ref : Inport  Port=4
  enable : Inport  Port=5
  Constant : Constant  Value=0
  Gain : Gain  Gain=-1
  Gain1 : Gain  Gain=1/500e-6
  Integrator1 : Integrator
  LPF : controls_element_lib/circuit_controls_A/LPF  SystemSampleTime=-1
  LPF1 : controls_element_lib/circuit_controls_A/LPF1  SystemSampleTime=-1
  Saturation Dynamic : simulink/Discontinuities/Saturation Dynamic  OutMin=[]  OutMax=[]  OutDataTypeStr=Inherit: Same as second input  OutDataType=fixdt(1, 16)  OutScaling=2^-10  DoSatur=off
  Sum : Sum  Inputs=|++
  Sum1 : Sum  Inputs=|+-
  Sum2 : Sum  Inputs=-+|
  Sum3 : Sum  Inputs=++|
  Sum6 : Sum  Inputs=|+-
  Switch : Switch  Criteria=u2 > Threshold
  kp : Gain  Gain=200
  kp_slow : Gain  Gain=2
  virtual damper : Subsystem
  v_bridge : Outport  VectorParamsAs1DForOutWhenUnconnected=on
  wires:
  LPF1/1 -> Sum3/1, virtual damper/1(v)
  Sum/1 -> Sum3/2
  Sum6/1 -> Switch/1
  LPF/1 -> Sum6/2
  Constant/1 -> Switch/3
  enable/1 -> Switch/2
  v_dc[3]/1 -> Gain/1, Saturation Dynamic/1
  Sum3/1 -> Saturation Dynamic/2
  v_ac/1 -> LPF1/1
  virtual damper/1(i_damp) -> Sum2/1
  i_ref/1 -> Sum2/2
  Switch/1 -> kp_slow/1, kp/1
  i_L/1 -> LPF/1
  Saturation Dynamic/1 -> v_bridge/1
  Sum2/1 -> Sum6/1
  kp/1 -> Sum/1
  Integrator1/1 -> Sum/2, Sum1/2
  Sum1/1 -> Gain1/1
  Gain1/1 -> Integrator1/1
  kp_slow/1 -> Sum1/1
  Gain/1 -> Saturation Dynamic/3

== system My_gfm_datacenter_BESS/Inverter Controller2/circuitControls_B (SST) ==
  i_ref : Inport
  enable : Inport  Port=2
  Constant : Constant  Value=0
  Switch : Switch  Criteria=u2 > Threshold
  ILoad : Outport  VectorParamsAs1DForOutWhenUnconnected=on
  wires:
  i_ref/1 -> Switch/1
  Constant/1 -> Switch/3
  enable/1 -> Switch/2
  Switch/1 -> ILoad/1

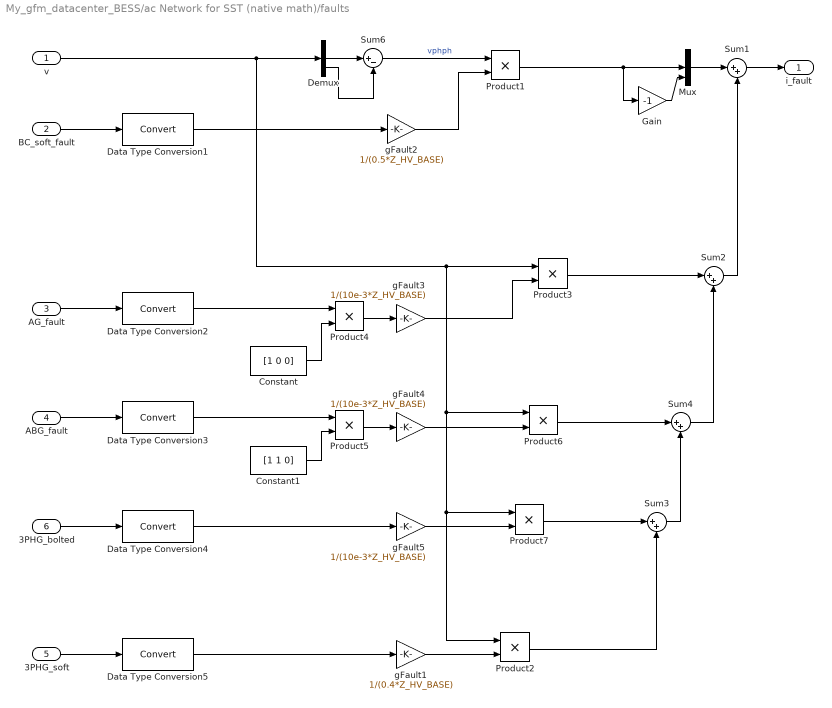
== system My_gfm_datacenter_BESS/ac Network for SST (native math)/faults ==
  v : Inport
  BC_soft_fault : Inport  Port=2
  AG_fault : Inport  Port=3
  ABG_fault : Inport  Port=4
  3PHG_soft : Inport  Port=5
  3PHG_bolted : Inport  Port=6
  Constant : Constant  Value=[1 0 0]
  Constant1 : Constant  Value=[1 1 0]
  Data Type Conversion{1..5} (5 alike) : DataTypeConversion
  Demux : Demux  Outputs=3
  Gain : Gain  Gain=-1
  Mux : Mux  Inputs=3
  Product{1..7} (7 alike) : Product
  Sum{1..4} (4 alike) : Sum  Inputs=|++
  Sum6 : Sum  Inputs=|+-
  gFault1 : Gain  Gain=1/(0.4*Z_HV_BASE)
  gFault2 : Gain  Gain=1/(0.5*Z_HV_BASE)
  gFault3 : Gain  Gain=1/(10e-3*Z_HV_BASE)
  gFault4 : Gain  Gain=1/(10e-3*Z_HV_BASE)
  gFault5 : Gain  Gain=1/(10e-3*Z_HV_BASE)
  i_fault : Outport  VectorParamsAs1DForOutWhenUnconnected=on
  wires:
  Product2/1 -> Sum3/2
  gFault1/1 -> Product2/2
  Sum1/1 -> i_fault/1
  Product1/1 -> Gain/1, Mux/2
  v/1 -> Demux/1, Product3/1, Product6/1, Product7/1, Product2/1
  Demux/3 -> Sum6/2
  Demux/2 -> Sum6/1
  Gain/1 -> Mux/3
  Sum6/1 -> Product1/1  "vphph"
  gFault2/1 -> Product1/2
  gFault3/1 -> Product3/2
  Mux/1 -> Sum1/1
  Product4/1 -> gFault3/1
  Constant/1 -> Product4/2
  Constant1/1 -> Product5/2
  Product5/1 -> gFault4/1
  Product3/1 -> Sum2/1
  gFault4/1 -> Product6/2
  gFault5/1 -> Product7/2
  BC_soft_fault/1 -> Data Type Conversion1/1
  AG_fault/1 -> Data Type Conversion2/1
  ABG_fault/1 -> Data Type Conversion3/1
  3PHG_bolted/1 -> Data Type Conversion4/1
  3PHG_soft/1 -> Data Type Conversion5/1
  Sum2/1 -> Sum1/2
  Product6/1 -> Sum4/1
  Sum4/1 -> Sum2/2
  Product7/1 -> Sum3/1
  Sum3/1 -> Sum4/2
  Data Type Conversion1/1 -> gFault2/1
  Data Type Conversion2/1 -> Product4/1
  Data Type Conversion3/1 -> Product5/1
  Data Type Conversion4/1 -> gFault5/1
  Data Type Conversion5/1 -> gFault1/1

== system My_gfm_datacenter_BESS/ac Network for SST (native math)/filter_caps ==
  i : Inport
  Gain1 : Gain  Gain=1/(0.03*C_MV_BASE)
  Integrator1 : Integrator
  v : Outport  VectorParamsAs1DForOutWhenUnconnected=on
  wires:
  Gain1/1 -> Integrator1/1
  Integrator1/1 -> v/1
  i/1 -> Gain1/1

== system My_gfm_datacenter_BESS/ac Network for SST (native math)/filter_inductors ==
  v : Inport
  en : Inport  Port=2
  Gain1 : Gain  Gain=1/(0.02*L_MV_BASE)
  Integrator1 : Integrator  ExternalReset=level
  NOT : Logic  Operator=NOT  IconShape=distinctive  AllPortsSameDT=off  OutDataTypeStr=boolean
  i : Outport  VectorParamsAs1DForOutWhenUnconnected=on
  wires:
  NOT/1 -> Integrator1/2
  v/1 -> Gain1/1
  Integrator1/1 -> i/1
  Gain1/1 -> Integrator1/1
  en/1 -> NOT/1

== system My_gfm_datacenter_BESS/ac Network for SST (native math)/solver_LPF ==
  In1 : Inport
  Gain : Gain  Gain=1/50e-6
  Integrator1 : Integrator
  Sum1 : Sum  Inputs=|+-
  Out1 : Outport  VectorParamsAs1DForOutWhenUnconnected=on
  wires:
  Gain/1 -> Integrator1/1
  Sum1/1 -> Gain/1
  Integrator1/1 -> Out1/1, Sum1/2
  In1/1 -> Sum1/1

== system My_gfm_datacenter_BESS/ac Network for SST (native math)/solver_LPF1 ==
  In1 : Inport
  Gain : Gain  Gain=1/1e-3
  Integrator1 : Integrator
  Sum1 : Sum  Inputs=|+-
  Out1 : Outport  VectorParamsAs1DForOutWhenUnconnected=on
  wires:
  In1/1 -> Sum1/1
  Integrator1/1 -> Sum1/2, Out1/1
  Sum1/1 -> Gain/1
  Gain/1 -> Integrator1/1

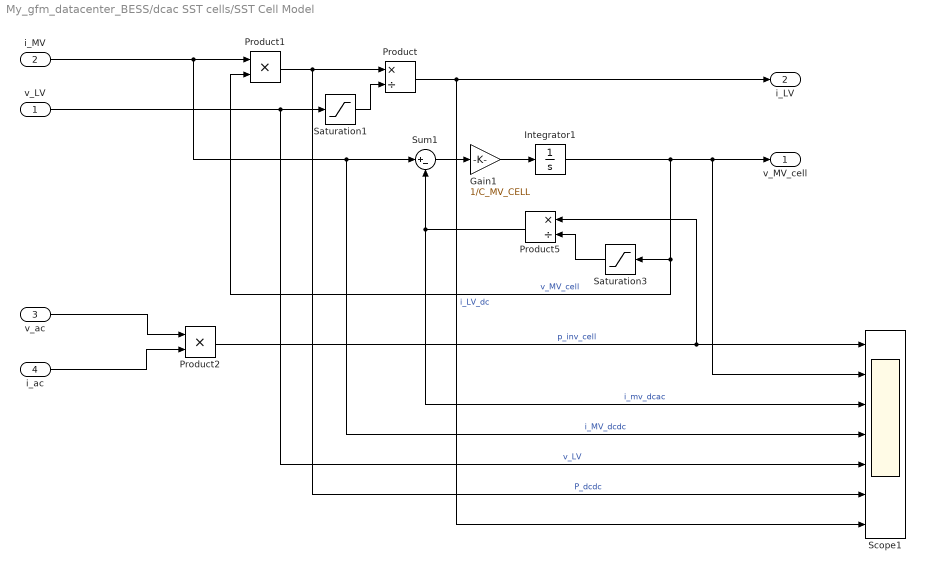
== system My_gfm_datacenter_BESS/dcac SST cells/SST Cell Model ==
  v_LV : Inport
  i_MV : Inport  Port=2
  v_ac : Inport  Port=3
  i_ac : Inport  Port=4
  Gain1 : Gain  Gain=1/C_MV_CELL
  Integrator1 : Integrator
  Product : Product  Inputs=*/
  Product1 : Product
  Product2 : Product
  Product5 : Product  Inputs=*/
  Saturation1 : Saturate  UpperLimit=inf  LowerLimit=50
  Saturation3 : Saturate  UpperLimit=inf  LowerLimit=500
  Scope1 : Scope  NumInputPorts=7
  Sum1 : Sum  Inputs=|+-
  v_MV_cell : Outport  VectorParamsAs1DForOutWhenUnconnected=on
  i_LV : Outport  Port=2  VectorParamsAs1DForOutWhenUnconnected=on
  wires:
  Saturation1/1 -> Product/2
  Product/1 -> Scope1/7, i_LV/1  "i_LV_dc"
  v_ac/1 -> Product2/1
  i_ac/1 -> Product2/2
  Product2/1 -> Product5/1, Scope1/1  "p_inv_cell"
  i_MV/1 -> Scope1/4, Sum1/1, Product1/1  "i_MV_dcdc"
  Sum1/1 -> Gain1/1
  Product1/1 -> Scope1/6, Product/1  "P_dcdc"
  Product5/1 -> Scope1/3, Sum1/2  "i_mv_dcac"
  Gain1/1 -> Integrator1/1
  v_LV/1 -> Scope1/5, Saturation1/1  "v_LV"
  Saturation3/1 -> Product5/2
  Integrator1/1 -> Product1/2, Saturation3/1, Scope1/2, v_MV_cell/1  "v_MV_cell"

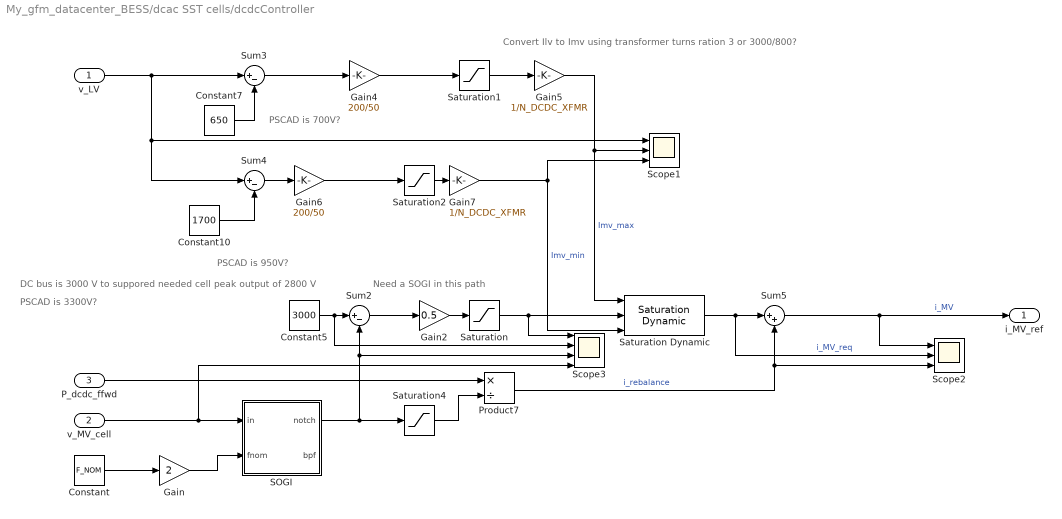
== system My_gfm_datacenter_BESS/dcac SST cells/dcdcController ==
  note: Convert Ilv to Imv using transformer turns ration 3 or 3000/800?
  note: DC bus is 3000 V to suppored needed cell peak output of 2800 V
  note: Need a SOGI in this path
  note: PSCAD is 3300V?
  note: PSCAD is 700V?
  note: PSCAD is 950V?
  v_LV : Inport
  v_MV_cell : Inport  Port=2
  P_dcdc_ffwd : Inport  Port=3
  Constant : Constant  Value=F_NOM
  Constant10 : Constant  Value=1700
  Constant5 : Constant  Value=3000
  Constant7 : Constant  Value=650
  Gain : Gain  Gain=2
  Gain2 : Gain  Gain=0.5
  Gain4 : Gain  Gain=200/50
  Gain5 : Gain  Gain=1/N_DCDC_XFMR
  Gain6 : Gain  Gain=200/50
  Gain7 : Gain  Gain=1/N_DCDC_XFMR
  Product7 : Product  Inputs=*/
  SOGI : Subsystem
  Saturation : Saturate  UpperLimit=IMV_MAX  LowerLimit=IMV_MIN
  Saturation Dynamic : simulink/Discontinuities/Saturation Dynamic  OutMin=[]  OutMax=[]  OutDataTypeStr=Inherit: Same as second input  OutDataType=fixdt(1, 16)  OutScaling=2^-10  DoSatur=off
  Saturation1 : Saturate  UpperLimit=ILV_MAX  LowerLimit=ILV_MIN
  Saturation2 : Saturate  UpperLimit=ILV_MAX  LowerLimit=ILV_MIN
  Saturation4 : Saturate  UpperLimit=inf  LowerLimit=2000
  Scope1 : Scope  NumInputPorts=3
  Scope2 : Scope  NumInputPorts=3
  Scope3 : Scope  NumInputPorts=4
  Sum2 : Sum  Inputs=|+-
  Sum3 : Sum  Inputs=|+-
  Sum4 : Sum  Inputs=|+-
  Sum5 : Sum  Inputs=|++
  i_MV_ref : Outport  VectorParamsAs1DForOutWhenUnconnected=on
  wires:
  Constant/1 -> Gain/1
  v_MV_cell/1 -> Scope3/4, SOGI/1(in)
  Gain/1 -> SOGI/2(fnom)
  Sum5/1 -> Scope2/1, i_MV_ref/1  "i_MV"
  Saturation4/1 -> Product7/2
  Sum3/1 -> Gain4/1
  Saturation2/1 -> Gain7/1
  Gain5/1 -> Saturation Dynamic/1, Scope1/2  "Imv_max"
  P_dcdc_ffwd/1 -> Product7/1
  Gain7/1 -> Saturation Dynamic/3, Scope1/3  "Imv_min"
  Product7/1 -> Scope2/3, Sum5/2  "i_rebalance"
  Gain6/1 -> Saturation2/1
  Sum4/1 -> Gain6/1
  Saturation Dynamic/1 -> Scope2/2, Sum5/1  "i_MV_req"
  Saturation1/1 -> Gain5/1
  Constant5/1 -> Scope3/2, Sum2/1
  v_LV/1 -> Scope1/1, Sum4/1, Sum3/1
  Constant7/1 -> Sum3/2
  Gain2/1 -> Saturation/1
  Saturation/1 -> Scope3/1, Saturation Dynamic/2
  Gain4/1 -> Saturation1/1
  SOGI/1(notch) -> Saturation4/1, Sum2/2, Scope3/3
  Sum2/1 -> Gain2/1
  Constant10/1 -> Sum4/2

== system My_gfm_datacenter_BESS/Datacenter plant controller (simplified)/Meter/PLL-analog ==
  ref : Inport
  Gain : Gain  Gain=3
  Gain2 : Gain  Gain=30
  Integrator : Integrator  LimitOutput=on  UpperSaturationLimit=5  LowerSaturationLimit=-5
  Product2 : Product
  Real-Imag to Complex : RealImagToComplex
  Saturation : Saturate  UpperLimit=5  LowerLimit=-5
  Sum of Elements : Sum  Inputs=+
  Sum1 : Sum  Inputs=|-+
  Sum2 : Sum  Inputs=|++
  Transfer Fcn : TransferFcn  Denominator=[0.02 1]
  fnom : Constant  Value=60
  oscillator : Subsystem
  freq : Outport  VectorParamsAs1DForOutWhenUnconnected=on
  osc : Outport  Port=2  VectorParamsAs1DForOutWhenUnconnected=on
  wires:
  Gain2/1 -> Integrator/1
  Integrator/1 -> Sum2/2
  Sum2/1 -> Sum1/1
  fnom/1 -> Sum1/2
  Product2/1 -> Sum of Elements/1
  oscillator/2(im) -> Product2/2, Real-Imag to Complex/2
  Transfer Fcn/1 -> Gain/1, Gain2/1
  Saturation/1 -> Sum2/1
  Gain/1 -> Saturation/1
  Sum1/1 -> freq/1, oscillator/1(f)
  ref/1 -> Product2/1
  oscillator/1(re) -> Real-Imag to Complex/1
  Real-Imag to Complex/1 -> osc/1
  Sum of Elements/1 -> Transfer Fcn/1

== system My_gfm_datacenter_BESS/Inverter Controller/BBU Charge Controller/SOGI ==
  in : Inport
  fnom : Inport  Port=2
  2pi : Gain  Gain=2*pi
  Integrator2 : Integrator
  Integrator3 : Integrator
  Product : Product
  Product1 : Product
  Sum4 : Sum  Inputs=|+-
  Sum5 : Sum  Inputs=|+-
  alpha : Gain  Gain=1/sqrt(2)
  notch : Outport  VectorParamsAs1DForOutWhenUnconnected=on
  bpf : Outport  Port=2  VectorParamsAs1DForOutWhenUnconnected=on
  wires:
  Product1/1 -> Integrator3/1
  Product/1 -> Integrator2/1
  2pi/1 -> Product/2, Product1/2
  Integrator3/1 -> Sum4/2
  Sum4/1 -> Product/1
  Sum5/1 -> notch/1, alpha/1
  alpha/1 -> Sum4/1
  Integrator2/1 -> bpf/1, Sum5/2, Product1/1
  fnom/1 -> 2pi/1
  in/1 -> Sum5/1

== system My_gfm_datacenter_BESS/Inverter Controller/dcVoltageRegulator_A/SOGI ==
  in : Inport
  fnom : Inport  Port=2
  2pi : Gain  Gain=2*pi
  Integrator2 : Integrator
  Integrator3 : Integrator
  Product : Product
  Product1 : Product
  Sum4 : Sum  Inputs=|+-
  Sum5 : Sum  Inputs=|+-
  alpha : Gain  Gain=1/sqrt(2)
  notch : Outport  VectorParamsAs1DForOutWhenUnconnected=on
  bpf : Outport  Port=2  VectorParamsAs1DForOutWhenUnconnected=on
  wires:
  Product1/1 -> Integrator3/1
  Product/1 -> Integrator2/1
  2pi/1 -> Product/2, Product1/2
  Integrator3/1 -> Sum4/2
  Sum4/1 -> Product/1
  Sum5/1 -> notch/1, alpha/1
  alpha/1 -> Sum4/1
  Integrator2/1 -> bpf/1, Sum5/2, Product1/1
  fnom/1 -> 2pi/1
  in/1 -> Sum5/1

== system My_gfm_datacenter_BESS/Inverter Controller1/circuitControls_B (SST)/virtual damper ==
  v : Inport
  1/tau_damp : Gain  Gain=1/250e-6
  Integrator : Integrator
  Sum : Sum  Inputs=|+-
  g_damp : Gain  Gain=1/(0.8*Z_INV_BASE)
  i_damp : Outport  VectorParamsAs1DForOutWhenUnconnected=on
  wires:
  g_damp/1 -> i_damp/1
  Sum/1 -> g_damp/1, 1/tau_damp/1
  v/1 -> Sum/1
  Integrator/1 -> Sum/2
  1/tau_damp/1 -> Integrator/1

== system My_gfm_datacenter_BESS/dcac SST cells/dcdcController/SOGI ==
  in : Inport
  fnom : Inport  Port=2
  2pi : Gain  Gain=2*pi
  Integrator2 : Integrator
  Integrator3 : Integrator
  Product : Product
  Product1 : Product
  Sum4 : Sum  Inputs=|+-
  Sum5 : Sum  Inputs=|+-
  alpha : Gain
  notch : Outport  VectorParamsAs1DForOutWhenUnconnected=on
  bpf : Outport  Port=2  VectorParamsAs1DForOutWhenUnconnected=on
  wires:
  in/1 -> Sum5/1
  fnom/1 -> 2pi/1
  Integrator2/1 -> Product1/1, Sum5/2, bpf/1
  alpha/1 -> Sum4/1
  Sum5/1 -> alpha/1, notch/1
  Sum4/1 -> Product/1
  Integrator3/1 -> Sum4/2
  2pi/1 -> Product1/2, Product/2
  Product/1 -> Integrator2/1
  Product1/1 -> Integrator3/1

== system My_gfm_datacenter_BESS/Datacenter plant controller (simplified)/Meter/PLL-analog/oscillator ==
  f : Inport
  2*pi : Gain  Gain=2*pi
  Cos : Trigonometry  Operator=cos
  Integrator : Integrator
  Rotation : Constant  Value=[0 -1 -2]*1/3
  Sin : Trigonometry
  Sum : Sum  Inputs=|++
  re : Outport  VectorParamsAs1DForOutWhenUnconnected=on
  im : Outport  Port=2  VectorParamsAs1DForOutWhenUnconnected=on
  wires:
  2*pi/1 -> Sin/1, Cos/1
  f/1 -> Integrator/1
  Cos/1 -> re/1
  Sin/1 -> im/1
  Sum/1 -> 2*pi/1
  Integrator/1 -> Sum/1
  Rotation/1 -> Sum/2
